simulink model "heater_driver_test"  (R2026a)
settings: Solver=ode23t  StopTime=4
libraries: fl_lib x10, nesl_utility x4, ee_lib x2
settings Model: Creator=Fufal Jigar  LastModifiedBy=Fufal Jigar

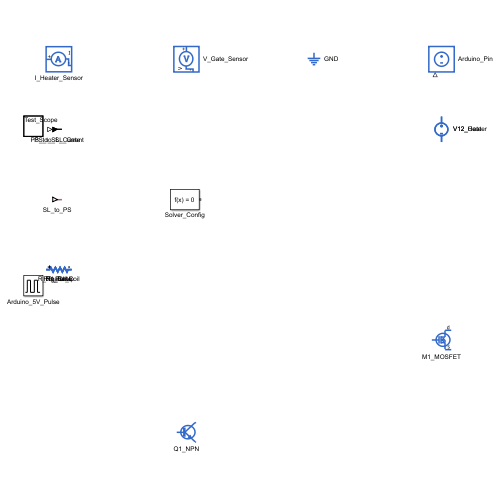
[thumbnail: Simulink's stored preview of the top-level diagram]
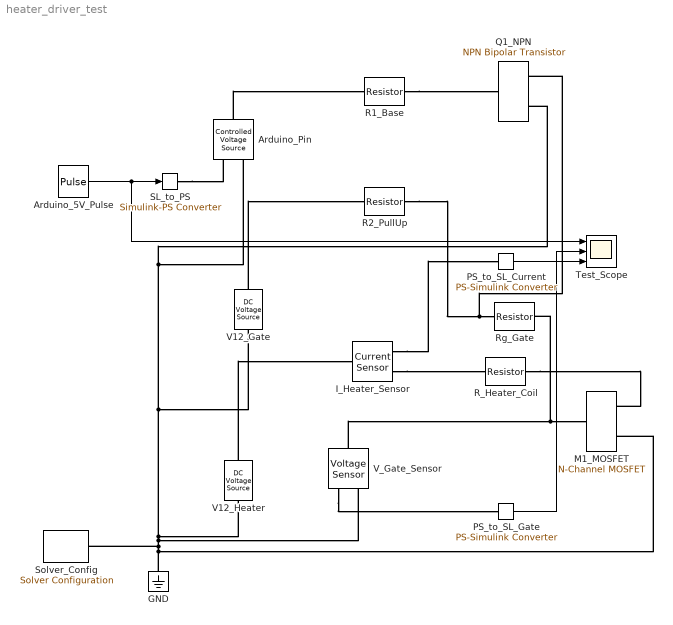
== system heater_driver_test ==
  Arduino_5V_Pulse : DiscretePulseGenerator  PulseType=Time based  Amplitude=5  PulseWidth=50  PhaseDelay=0.5
  Arduino_Pin : fl_lib/Electrical/Electrical Sources/Controlled Voltage Source
  GND : fl_lib/Electrical/Electrical Elements/Electrical Reference
  I_Heater_Sensor : fl_lib/Electrical/Electrical Sensors/Current Sensor
  M1_MOSFET : ee_lib/Semiconductors & Converters/N-Channel MOSFET  paramTerminal=ee.enum.mosfet.numberOfTerminals.three  parameterization=ee.enum.mosfet.parameterization.datasheet  Beta=5.0 A/V^2  Rds=0.025 Ohm  Id=6.0 A  Vgs=10 V  Vth=1.7 V  Vth0=1.7 V  lam=0 1/V  gamma_vth=0.5 V^(1/2)  phib=0.5 V  Vth1=1.9071 V  Vbs1=-1 V  Vth2=2.066 V  Vbs2=-2 V  Tmeas=25 degC  Vgs_vec=[-1, -.5, 2, 3, 4, 5] V  Vds_vec=[0, 2, 4, 8, 12, 16, 20] V  Vbs_vec=[0, -4, -6, -12] V  T_vec=[25, 125] degC  Vth_vec=[.4, 1.2, 1.4, 1.45] V  Vth_mat=[.4, .35; 1.2, 1.15; 1.4, 1.35; 1.45, 1.4] V  Ids_mat=[0, 0, 0, 0, 0, 0, 0; 0, 0, 0, 0, 0, 0, 0; 0, .003, .0038, .0043, .0046, .0048, .0049; 0, .0055, .008, .009, .0095, .01, .0101; 0, .0115, .016, .018, .019, .0195, .02; 0, .0152, .0225, .0265, .028, .0295, .03] A  Ids_mat0=[0, 0, 0, 0, 0, 0, 0; 0, 0, 0, 0, 0, 0, 0; 0, .003, .0038, .0043, .0046, .0048, .0049; 0, .0055, .008, .009, .0095, .01, .0101; 0, .0115, .016, .018, .019, .0195, .02; 0, .0152, .0225, .0265, .028, .0295, .03] A  Ids_mat_3D=zeros(6, 7, 2) A  Ids_mat_3D0=zeros(6, 7, 2) A  IV_table_symmetry=ee.enum.mosfet.symmetricNIV.no  RS=0.0001 Ohm  RD=0.01 Ohm  RB=0.001 Ohm  LeadRs=0 Ohm  LeadRd=0 Ohm  LeadRg=0 Ohm  LeadRb=0 Ohm  LS=0 nH  LD=0 nH  LG=0 nH  LB=0 nH  C_param=ee.enum.mosfet.capacitanceParam.fixedciss  C_GS=270 pF  C_GD=80 pF  C_GB=0 pF  C_DS=0 pF  C_iss=350 pF  C_rss=80 pF  C_oss=0 pF  C_iss_vec=[720, 700, 590, 470, 390, 310] pF  C_rss_vec=[450, 400, 300, 190, 95, 55] pF  C_oss_vec=[900, 810, 690, 420, 270, 170] pF  C_GS_vec=[270, 300, 290, 280, 295, 255] pF  C_GD_vec=[450, 400, 300, 190, 95, 55] pF  C_GB_vec=[270, 300, 290, 280, 295, 255] pF  C_Vgs_vec=0 V  C_DS_vec=[450, 410, 390, 230, 175, 115] pF  C_Vds_vec=[.1, .3, 1, 3, 10, 30] V  V_GS_for_cap_data=0 V  charge_linearity_param=ee.enum.mosfet.cgdLinearity.constant  C_OX=200 pF  V_C_OX=-0.5 V  charge_linearity_param_vgb=ee.enum.mosfet.cgbLinearity.instantly  charge_linearity_param_with_vgb=ee.enum.mosfet.cgbLinearityWithSeparateCgb.instantly  Di_param=ee.enum.mosfet.diodeParam.no  IsDiode=1e-12 A  Vbi=0.6 V  n=1  Cj0Diode=0 pF  TT=50e-9 s  Tmeas_dio=25 degC  TableTypeNoT=ee.enum.mosfet.tableType.IfMat  TableType=ee.enum.diode.tableType.IfMat  IfVec=[.07, .12, .19, 1.75, 4.24, 7.32, 11.2] A  IfMat=[.07, .12, .19, 1.75, 4.24, 7.32, 11.2; .16, .3, .72, 2.14, 4.02, 6.35, 9.12] A  VfVecV=[.9, 1.15, 1.25, 1.5, 1.75, 2.17, 2.6, 2.85] V  VfMatV=[.9, 1.15, 1.25, 1.5, 1.75, 2.17, 2.6, 2.85; .58, .68, .75, 1.1, 1.38, 1.77, 2.27, 2.7] V  TjVec=[25, 125] degC  VfVec=[.5, .7, .9, 1.3, 1.7, 2.1, 2.5] V  IfVecV=[.1, .2, .5, 1, 2, 4, 7, 10] A  diode_Goff=1e-12 1/Ohm  prmDatasheet=ee.enum.temperatureParameterization.none  prmEquCoeff=ee.enum.temperatureParameterization.none  dVth_dT=-6 mV/K  dVth0_dT=-6 mV/K  Rds_T2=0.037 Ohm  BEXDatasheet=-1.5  BEXEquCoeff=-1.5  etaisDatasheet=3  etaisEquCoeff=3  Tmeas2=125 degC  etaisTabulated=3  TdeviceDatasheet=25 degC  TdeviceEquCoeff=25 degC  TdeviceTabulated=25 degC  i_g_specify=off  i_g_priority=None  i_g=0 A  i_g_nominal_specify=off  i_g_nominal_value=1  i_g_nominal_unit=A  i_d_specify=off  i_d_priority=None  i_d=0 A  i_d_nominal_specify=off  i_d_nominal_value=1  i_d_nominal_unit=A  i_b_specify=off  i_b_priority=None  i_b=0 A  i_b_nominal_specify=off  i_b_nominal_value=1  i_b_nominal_unit=A  voltage_gs_specify=off  voltage_gs_priority=None  voltage_gs=0 V  voltage_gs_nominal_specify=off  voltage_gs_nominal_value=1  voltage_gs_nominal_unit=V  voltage_ds_specify=off  voltage_ds_priority=None  voltage_ds=0 V  voltage_ds_nominal_specify=off  voltage_ds_nominal_value=1  voltage_ds_nominal_unit=V  voltage_bs_specify=off  voltage_bs_priority=None  voltage_bs=0 V  voltage_bs_nominal_specify=off  voltage_bs_nominal_value=1  voltage_bs_nominal_unit=V  v_Cgs_specify=off  v_Cgs_priority=High  v_Cgs=0 V  v_Cgs_nominal_specify=off  v_Cgs_nominal_value=1  v_Cgs_nominal_unit=V  v_Cds_specify=off  v_Cds_priority=High  v_Cds=0 V  v_Cds_nominal_specify=off  v_Cds_nominal_value=1  v_Cds_nominal_unit=V  v_Cbs_specify=off  v_Cbs_priority=High  v_Cbs=0 V  v_Cbs_nominal_specify=off  v_Cbs_nominal_value=1  v_Cbs_nominal_unit=V  thermal_network_parameterization=ee.enum.thermalNetworkTopology.junctionCase  Rth=[0, 10] K/W  Rth_Cauer=[1, 3, 10] K/W  Rth_Foster=[.08, .14, .22, .16] K/W  thermal_mass_parameterization=ee.enum.thermalNetwork.timeconstant  thermal_mass=[0, 1] J/K  thermal_mass_Cauer=[.1, .3, 1] J/K  thermal_mass_Foster=[.001, .005, .05, .5] J/K  thermal_time_constant=[0, 10] s  thermal_time_constant_Cauer=[1, 3, 10] s  thermal_time_constant_Foster=[7e-05, .0007, .01, .08] s  thermal_mass_initial_temperatures=[25, 25] degC  thermal_mass_initial_temperatures_Cauer=[25, 25, 25] degC  Tvec_initial_Foster=[25, 25, 25, 25] degC  betaref=18 A/V^2  Vfbref=-1.1 V  gamma=3.5 V^(1/2)  phib2ref=1 V  thesatref=0.4 1/V  alpha=0  Vp=5e-2 V  thesrref=0 1/V  m=8  Tref=25 degC  Rsref=2e-3 Ohm  Rdref=0.17 Ohm  Rgref=8.4 Ohm  Rbref=2e-3 Ohm  Cox=1500 pF  Cgso=100 pF  Cgdo=14 pF  Isref=5.2e-13 A  Cj0=480 pF  Tprm=ee.enum.temperatureParameterization.none  etabet=1.3  Stvfb=5e-4 V/K  Stphib=-8.5e-4 V/K  etasat=1.04  etasr=0.65  etar=0.95  etais=3  Tsim=25 degC  Ig_specify=off  Ig_priority=None  Ig=0 A  Ig_nominal_specify=off  Ig_nominal_value=1  Ig_nominal_unit=nA  Ids_specify=off  Ids_priority=None  Ids=0 A  Ids_nominal_specify=off  Ids_nominal_value=1  Ids_nominal_unit=A  Ib_specify=off  Ib_priority=None  Ib=0 A  Ib_nominal_specify=off  Ib_nominal_value=1  Ib_nominal_unit=uA  V_gs_specify=off  V_gs_priority=None  V_gs=0 V  V_gs_nominal_specify=off  V_gs_nominal_value=1  V_gs_nominal_unit=V  V_ds_specify=off  V_ds_priority=None  V_ds=0 V  V_ds_nominal_specify=off  V_ds_nominal_value=1  V_ds_nominal_unit=V  V_bs_specify=off  V_bs_priority=None  V_bs=0 V  V_bs_nominal_specify=off  V_bs_nominal_value=1  V_bs_nominal_unit=V  QGoverCox_specify=off  QGoverCox_priority=None  QGoverCox=0 V  QGoverCox_nominal_specify=off  QGoverCox_nominal_value=1  QGoverCox_nominal_unit=V  QDoverCox_specify=off  QDoverCox_priority=None  QDoverCox=0 V  QDoverCox_nominal_specify=off  QDoverCox_nominal_value=1  QDoverCox_nominal_unit=V  QBoverCox_specify=off  QBoverCox_priority=None  QBoverCox=0 V  QBoverCox_nominal_specify=off  QBoverCox_nominal_value=1  QBoverCox_nominal_unit=V  T0=[25, 25] degC  T0_Cauer=[25, 25, 25] degC
  PS_to_SL_Current : nesl_utility/PS-Simulink Converter  PhysicalDomain=network_engine_domain  SubClassName=ps_output  LeftPortType=input  RightPortType=output  PseudoPeriodic=off  Frequencies=[]  VectorFormat=inherit  Unit=inherit  AffineConversion=off
  PS_to_SL_Gate : nesl_utility/PS-Simulink Converter  PhysicalDomain=network_engine_domain  SubClassName=ps_output  LeftPortType=input  RightPortType=output  PseudoPeriodic=off  Frequencies=[]  VectorFormat=inherit  Unit=inherit  AffineConversion=off
  Q1_NPN : ee_lib/Semiconductors & Converters/NPN Bipolar Transistor  parameterization=1  BF=100  IS=1e-14 A  VAF=200 V  hfe=100  hoe=50e-6 1/Ohm  Ic_h=1 mA  Vce_h=5 V  V1=0.55 V  I1=0.5 mA  BR=1  Tmeas=25 degC  RC=0.01 Ohm  RE=1e-4 Ohm  RB=1 Ohm  C_BC=5 pF  C_BE=5 pF  TF=0 us  TR=0 us  prmDatasheet=1  prmEquCoeff=1  hfe_T2=125  XTB=0  V1_T2=0.45 V  I1_T2=0.5 mA  Tmeas2=125 degC  EG=1.11 eV  XTI=3  TdeviceDatasheet=25 degC  TdeviceEquCoeff=25 degC  ec=1  ib_specify=off  ib_priority=None  ib=0 A  ib_nominal_specify=off  ib_nominal_value=1  ib_nominal_unit=A  ic_specify=off  ic_priority=None  ic=0 A  ic_nominal_specify=off  ic_nominal_value=1  ic_nominal_unit=A  vce_specify=off  vce_priority=None  vce=0 V  vce_nominal_specify=off  vce_nominal_value=1  vce_nominal_unit=V  vbe_specify=off  vbe_priority=None  vbe=0 V  vbe_nominal_specify=off  vbe_nominal_value=1  vbe_nominal_unit=V  Qbc_specify=off  Qbc_priority=High  Qbc=0 C  Qbc_nominal_specify=off  Qbc_nominal_value=1  Qbc_nominal_unit=uC  Qbe_specify=off  Qbe_priority=High  Qbe=0 C  Qbe_nominal_specify=off  Qbe_nominal_value=1  Qbe_nominal_unit=uC  thermal_network_parameterization=ee.enum.thermalNetworkTopology.junctionCase  Rth=[0, 10] K/W  Rth_Cauer=[1, 3, 10] K/W  Rth_Foster=[.08, .14, .22, .16] K/W  thermal_mass_parameterization=ee.enum.thermalNetwork.timeconstant  thermal_mass=[0, 1] J/K  thermal_mass_Cauer=[.1, .3, 1] J/K  thermal_mass_Foster=[.001, .005, .05, .5] J/K  thermal_time_constant=[0, 10] s  thermal_time_constant_Cauer=[1, 3, 10] s  thermal_time_constant_Foster=[7e-05, .0007, .01, .08] s  thermal_mass_initial_temperatures=[25, 25] degC  thermal_mass_initial_temperatures_Cauer=[25, 25, 25] degC  Tvec_initial_Foster=[25, 25, 25, 25] degC
  R1_Base : fl_lib/Electrical/Electrical Elements/Resistor  R=2200 Ohm  i_specify=off  i_priority=None  i=0 A  i_nominal_specify=off  i_nominal_value=1  i_nominal_unit=A  v_specify=off  v_priority=None  v=0 V  v_nominal_specify=off  v_nominal_value=1  v_nominal_unit=V
  R2_PullUp : fl_lib/Electrical/Electrical Elements/Resistor  R=2200 Ohm  i_specify=off  i_priority=None  i=0 A  i_nominal_specify=off  i_nominal_value=1  i_nominal_unit=A  v_specify=off  v_priority=None  v=0 V  v_nominal_specify=off  v_nominal_value=1  v_nominal_unit=V
  R_Heater_Coil : fl_lib/Electrical/Electrical Elements/Resistor  R=10 Ohm  i_specify=off  i_priority=None  i=0 A  i_nominal_specify=off  i_nominal_value=1  i_nominal_unit=A  v_specify=off  v_priority=None  v=0 V  v_nominal_specify=off  v_nominal_value=1  v_nominal_unit=V
  Rg_Gate : fl_lib/Electrical/Electrical Elements/Resistor  R=10 Ohm  i_specify=off  i_priority=None  i=0 A  i_nominal_specify=off  i_nominal_value=1  i_nominal_unit=A  v_specify=off  v_priority=None  v=0 V  v_nominal_specify=off  v_nominal_value=1  v_nominal_unit=V
  SL_to_PS : nesl_utility/Simulink-PS Converter  PhysicalDomain=network_engine_domain  SubClassName=ps_input  LeftPortType=input  RightPortType=output  PseudoPeriodic=off  Frequencies=[]  NoiseDistribution=none  NoiseParameters=[]  Unit=1  AffineConversion=off  FilteringAndDerivatives=provide  SimscapeFilterOrder=1  InputFilterTimeConstant=0.001  UdotUserProvided=0
  Solver_Config : nesl_utility/Solver Configuration  PhysicalDomain=network_engine_domain  SubClassName=solver  LeftPortType=input  RightPortType=generic  Tones=[]  Harmonics=[]  SimulateNoise=off  Profile=off  UseLocalSampling=off  EnableSwitchedLinearOptims=on  FrequencyDomain=off  UseCCode=off  RelTol=0.001  AbsTol=0.001  MinStep=1e-09  ToWorkspace=off  RevertToSquareIcSolve=off  NumHomotopyIterations=100  PhasorMode=off  PhasorModeNumHarmonics=1  ConsistencySolver=NEWTON_XTOL_AFTER_FTOL  CanonicalOrdering=CANONICAL  OptimizeIntermediates=OPTIMIZED  IndexReductionMethod=DerivativeReplacement  DoDC=off  ResidualTolerance=1e-09  ConsistencyTolSource=GLOBAL  ConsistencyAbsTol=0.001  ConsistencyRelTol=0.001  ConsistencyTolFactor=0.001  UseLocalSolver=off  LocalSolverChoice=NE_BACKWARD_EULER_ADVANCER  ResolveIndetEquations=on  FunctionEvalNumThread=1  LocalSolverSampleTime=0.001  DoFixedCost=off  MaxNonlinIter=3  MaxModeIter=2  ComputeImpulses=off  ImpulseIterations=2  LinearAlgebra=auto  LinearAlgebraNumThread=0  EquationFormulation=NE_TIME_EF  DelaysMemoryBudget=1024  AutomaticFiltering=on  FilteringTimeConstant=0.001  PartitionStorageMethod=AS_NEEDED  PartitionMemoryBudget=1024  PartitionMethod=ROBUST  MultibodyUseLocalSolver=off  MultibodyLocalSolverChoice=ODE1  MultibodyLocalSolverSampleTime=0.001
  Test_Scope : Scope  NumInputPorts=3
  V12_Gate : fl_lib/Electrical/Electrical Sources/DC Voltage Source  v0=12 V
  V12_Heater : fl_lib/Electrical/Electrical Sources/DC Voltage Source  v0=12 V
  V_Gate_Sensor : fl_lib/Electrical/Electrical Sensors/Voltage Sensor
  wires:
  Arduino_5V_Pulse/1 -> Test_Scope/1, SL_to_PS/1
  PS_to_SL_Current/1 -> Test_Scope/3
  PS_to_SL_Gate/1 -> Test_Scope/2
  connections:
  Arduino_Pin/LConn1 -- R1_Base/LConn1
  SL_to_PS/RConn1 -- Arduino_Pin/RConn1
  V_Gate_Sensor/LConn1 -- M1_MOSFET/LConn1 -- Rg_Gate/RConn1
  V_Gate_Sensor/RConn1 -- PS_to_SL_Gate/LConn1
  GND/LConn1 -- Arduino_Pin/RConn2 -- Q1_NPN/RConn2 -- V12_Gate/RConn1 -- V12_Heater/RConn1 -- V_Gate_Sensor/RConn2 -- Solver_Config/RConn1 -- M1_MOSFET/RConn2
  R1_Base/RConn1 -- Q1_NPN/LConn1
  V12_Gate/LConn1 -- R2_PullUp/LConn1
  V12_Heater/LConn1 -- I_Heater_Sensor/LConn1
  R2_PullUp/RConn1 -- Q1_NPN/RConn1 -- Rg_Gate/LConn1
  I_Heater_Sensor/RConn1 -- PS_to_SL_Current/LConn1
  I_Heater_Sensor/RConn2 -- R_Heater_Coil/LConn1
  R_Heater_Coil/RConn1 -- M1_MOSFET/RConn1
